simulink model "Safebeat_v1"  (R2019a)
settings: Solver=FixedStepDiscrete  StartTime=0.0  StopTime=10.0  FixedStep=1/360  RelTol=1e-3
libraries: simulink x2, dsparch4 x1
settings Model: Creator=Admin  LastModifiedBy=Admin

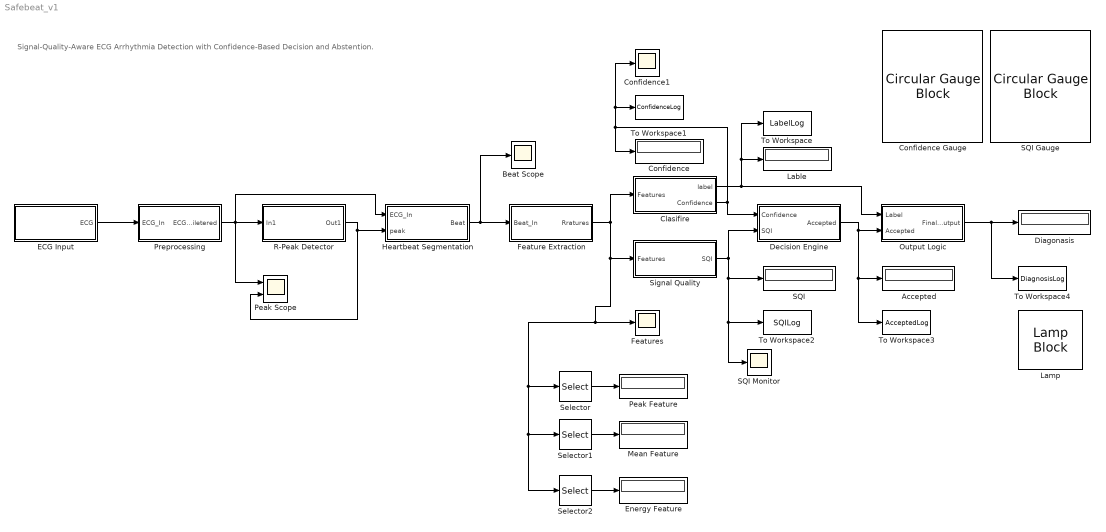
== system Safebeat_v1 ==
  note: Signal-Quality-Aware ECG Arrhythmia Detection with Confidence-Based Decision and Abstention.
  Accepted : Display
  Beat Scope : Scope
  Clasifire : Subsystem
  Confidence : Display
  Confidence Gauge : CircularGaugeBlock  ScaleMax=1
  Confidence1 : Scope
  Decision Engine : Subsystem
  "Diagonasis " : Display
  ECG Input : Subsystem
  "Energy Feature " : Display
  Feature Extraction : Subsystem
  Features : Scope
  Heartbeat Segmentation : Subsystem
  Lable : Display
  Lamp : LampBlock
  Mean Feature : Display
  Output Logic : Subsystem
  Peak Feature : Display
  Peak Scope : Scope  NumInputPorts=2
  Preprocessing : Subsystem
  R-Peak Detector : Subsystem
  SQI : Display
  SQI Gauge : CircularGaugeBlock  ScaleMax=1
  SQI Monitor : Scope
  Selector : Selector  InputPortWidth=3  IndexOptions=Index vector (dialog)  Indices=1  OutputSizes=1
  Selector1 : Selector  InputPortWidth=3  IndexOptions=Index vector (dialog)  Indices=2  OutputSizes=1
  Selector2 : Selector  InputPortWidth=3  IndexOptions=Index vector (dialog)  Indices=3  OutputSizes=1
  Signal Quality : Subsystem
  To Workspace : ToWorkspace  VariableName=LabelLog  SampleTime=-1
      settings: Save2DSignal=2-D array (concatenate along first dimension)
  To Workspace1 : ToWorkspace  VariableName=ConfidenceLog  SampleTime=-1
      settings: Save2DSignal=2-D array (concatenate along first dimension)
  To Workspace2 : ToWorkspace  VariableName=SQILog  SampleTime=-1
      settings: Save2DSignal=2-D array (concatenate along first dimension)
  To Workspace3 : ToWorkspace  VariableName=AcceptedLog  SampleTime=-1
      settings: Save2DSignal=2-D array (concatenate along first dimension)
  To Workspace4 : ToWorkspace  VariableName=DiagnosisLog  SampleTime=-1
      settings: Save2DSignal=2-D array (concatenate along first dimension)
  wires:
  Preprocessing/1(ECG_Filetered) -> Peak Scope/1, R-Peak Detector/1(In1), Heartbeat Segmentation/1(ECG_In)
  Heartbeat Segmentation/1("Beat ") -> Beat Scope/1, Feature Extraction/1(Beat_In)
  Feature Extraction/1(Rratures) -> Selector2/1, Selector1/1, Selector/1, Features/1, Signal Quality/1(Features), Clasifire/1(Features)
  Clasifire/2(Confidence) -> Confidence/1, Confidence1/1, To Workspace1/1, Decision Engine/1(Confidence)
  Clasifire/1(label) -> Output Logic/1(Label), Lable/1, To Workspace/1
  Signal Quality/1(SQI) -> Decision Engine/2(SQI), To Workspace2/1, SQI Monitor/1, SQI/1
  Decision Engine/1(Accepted) -> Output Logic/2(Accepted), To Workspace3/1, Accepted/1
  Output Logic/1(FinalOutput) -> To Workspace4/1, "Diagonasis "/1
  ECG Input/1(ECG) -> Preprocessing/1(ECG_In)
  R-Peak Detector/1(Out1) -> Peak Scope/2, Heartbeat Segmentation/2(peak)
  Selector/1 -> Peak Feature/1
  Selector1/1 -> Mean Feature/1
  Selector2/1 -> "Energy Feature "/1

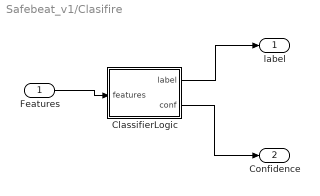
== system Safebeat_v1/Clasifire ==
  Features : Inport
  ClassifierLogic : MATLAB Function  TreatAsAtomicUnit=on
  label : Outport
  Confidence : Outport  Port=2
  wires:
  ClassifierLogic/1(label) -> label/1
  Features/1 -> ClassifierLogic/1(features)
  ClassifierLogic/2(conf) -> Confidence/1

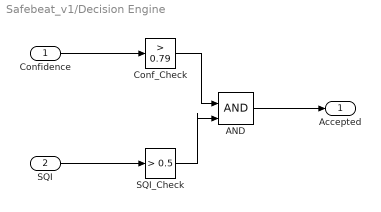
== system Safebeat_v1/Decision Engine ==
  Confidence : Inport
  SQI : Inport  Port=2
  AND : Logic  IconShape=distinctive  AllPortsSameDT=off  OutDataTypeStr=boolean
  Conf_Check : simulink/Logic and Bit Operations/Compare To Constant  relop=>  const=0.79  OutDataTypeStr=boolean
  SQI_Check : simulink/Logic and Bit Operations/Compare To Constant  relop=>  const=0.5  OutDataTypeStr=boolean
  Accepted : Outport
  wires:
  Confidence/1 -> Conf_Check/1
  Conf_Check/1 -> AND/1
  SQI/1 -> SQI_Check/1
  SQI_Check/1 -> AND/2
  AND/1 -> Accepted/1

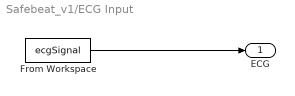
== system Safebeat_v1/ECG Input ==
  From Workspace : FromWorkspace  VariableName=ecgSignal  SampleTime=0
  ECG : Outport
  wires:
  From Workspace/1 -> ECG/1

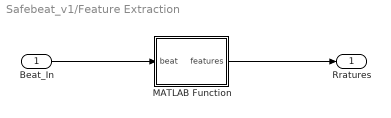
== system Safebeat_v1/Feature Extraction ==
  Beat_In : Inport
  MATLAB Function : MATLAB Function  TreatAsAtomicUnit=on
  Rratures : Outport
  wires:
  MATLAB Function/1(features) -> Rratures/1
  Beat_In/1 -> MATLAB Function/1(beat)

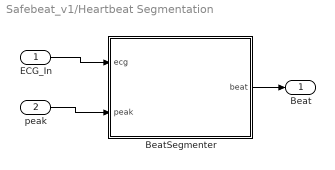
== system Safebeat_v1/Heartbeat Segmentation ==
  ECG_In : Inport
  peak : Inport  Port=2
  BeatSegmenter : MATLAB Function  TreatAsAtomicUnit=on
  "Beat " : Outport
  wires:
  ECG_In/1 -> BeatSegmenter/1(ecg)
  BeatSegmenter/1(beat) -> "Beat "/1
  peak/1 -> BeatSegmenter/2(peak)

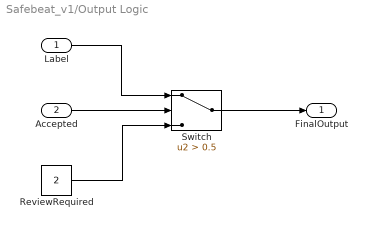
== system Safebeat_v1/Output Logic ==
  Label : Inport
  Accepted : Inport  Port=2
  ReviewRequired : Constant  Value=2
  Switch : Switch  Criteria=u2 > Threshold  Threshold=0.5
  FinalOutput : Outport
  wires:
  Switch/1 -> FinalOutput/1
  Label/1 -> Switch/1
  Accepted/1 -> Switch/2
  ReviewRequired/1 -> Switch/3

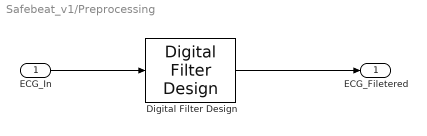
== system Safebeat_v1/Preprocessing ==
  ECG_In : Inport
  Digital Filter Design : dsparch4/Digital Filter Design  mwdsp_browser_bugfix_var=off
  ECG_Filetered : Outport
  wires:
  ECG_In/1 -> Digital Filter Design/1
  Digital Filter Design/1 -> ECG_Filetered/1

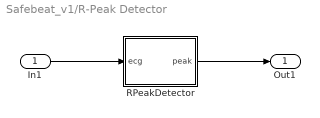
== system Safebeat_v1/R-Peak Detector ==
  In1 : Inport
  RPeakDetector : MATLAB Function  TreatAsAtomicUnit=on
  Out1 : Outport
  wires:
  In1/1 -> RPeakDetector/1(ecg)
  RPeakDetector/1(peak) -> Out1/1

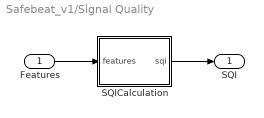
== system Safebeat_v1/Signal Quality ==
  Features : Inport
  SQICalculation : MATLAB Function  TreatAsAtomicUnit=on
  SQI : Outport
  wires:
  Features/1 -> SQICalculation/1(features)
  SQICalculation/1(sqi) -> SQI/1

== matlab function Safebeat_v1/Feature Extraction/MATLAB Function ==
  data: beat input; features output size=[3 1]
function features = extractFeatures(beat)

peakAmp = max(abs(beat));

meanAmp = mean(abs(beat));

energy = sum(beat.^2);

features = [peakAmp; meanAmp; energy];

end

== matlab function Safebeat_v1/Heartbeat Segmentation/BeatSegmenter ==
  data: ecg input; beat output size=[110 1]; peak input
function beat = BeatSegmenter(ecg, peak)

persistent buffer

if isempty(buffer)
    buffer = zeros(110,1);
end

buffer(1:end-1) = buffer(2:end);
buffer(end) = ecg;

% Debug version
beat = buffer;

end

== matlab function Safebeat_v1/R-Peak Detector/RPeakDetector ==
  data: ecg input; peak output
function peak = RPeakDetector(ecg)

persistent prev1 prev2

if isempty(prev1)
    prev1 = 0;
    prev2 = 0;
end

peak = 0;

sig = abs(ecg);

if (prev1 > prev2) && ...
   (prev1 > sig) && ...
   (prev1 > 0.5)

    peak = 1;
end

prev2 = prev1;
prev1 = sig;

end

== matlab function Safebeat_v1/Signal Quality/SQICalculation ==
  data: features input; sqi output double size=1
function sqi = calcSQI(features)

meanAmp = features(2);

sqi = exp(-meanAmp/100);

end

== matlab function Safebeat_v1/Clasifire/ClassifierLogic ==
  data: features input; label output double size=1; conf output double size=1
function [label, conf] = classify(features)

peakAmp = features(1);
meanAmp = features(2);
energy  = features(3);

score = 0;

if peakAmp > 1.5
    score = score + 1;
end

if meanAmp > 0.3
    score = score + 1;
end

if energy > 300000
    score = score + 1;
end

if score >= 2
    label = 1;    % PVC
    conf = 0.90;
else
    label = 0;    % Normal
    conf = 0.80;
end

end
